simulink model "Caldeira_Controle"  (R2024a)
settings: Solver=ode45  StartTime=0.0  StopTime=260  MaxStep=0.02  RelTol=1e-5
PreLoadFcn:
  | if ~exist('cfg_vap','var') || ~exist('cfg_niv','var'), config_caldeira; end
InitFcn:
  | if ~exist('cfg_vap','var') || ~exist('cfg_niv','var'), config_caldeira; end
settings Model: Creator=Vinicius  LastModifiedBy=Vinicius

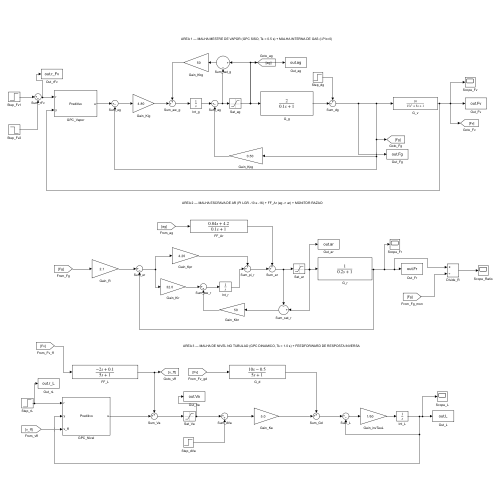
[thumbnail: Simulink's stored preview of the top-level diagram]
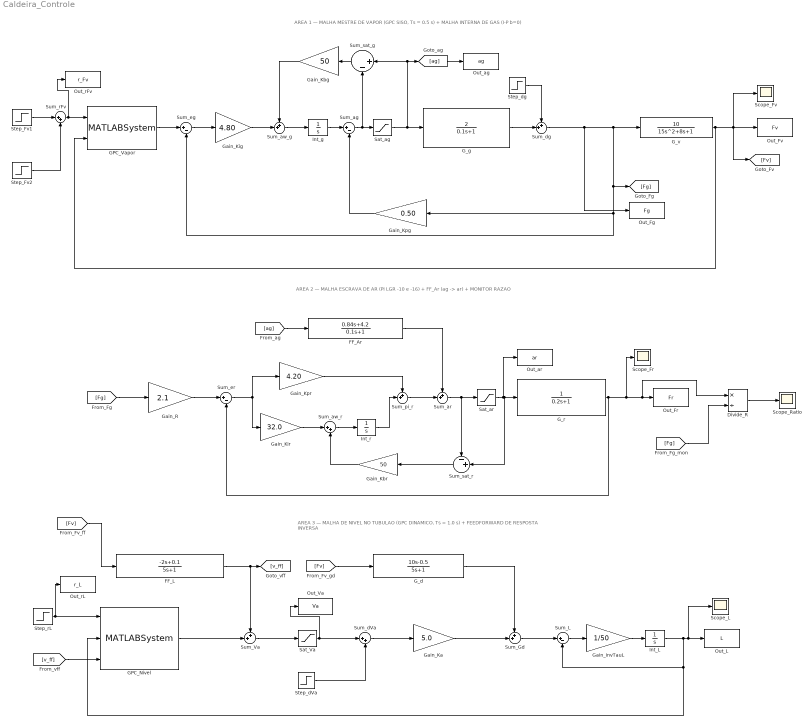
== system Caldeira_Controle ==
  note: AREA 1 — MALHA MESTRE DE VAPOR (GPC SISO, Ts = 0.5 s) + MALHA INTERNA DE GAS (I-P b=0)
  note: AREA 2 — MALHA ESCRAVA DE AR (PI LGR -10 e -16) + FF_Ar (ag -> ar) + MONITOR RAZAO
  note: AREA 3 — MALHA DE NIVEL NO TUBULAO (GPC DINAMICO, Ts = 1.0 s) + FEEDFORWARD DE RESPOSTA INVERSA
  Divide_R : Product  Inputs=*/
  FF_Ar : TransferFcn  Numerator=[0.84 4.2]  Denominator=[0.1 1]
  FF_L : TransferFcn  Numerator=[-2 0.1]  Denominator=[5 1]
  GPC_Nivel : MATLABSystem  System=ControladorPreditivoDin  cfg=cfg_niv
      mask Type: ControladorPreditivoDin
      mask Display:
      | disp('Preditivo');
      | port_label('input',1,'r');
      | port_label('input',2,'y');
      | port_label('input',3,'v_ff');
      | port_label('output',1,'u');
  GPC_Vapor : MATLABSystem  System=ControladorPreditivo  cfg=cfg_vap
      mask Type: ControladorPreditivo
      mask Display:
      | disp('Preditivo');
      | port_label('input',1,'r');
      | port_label('input',2,'y');
      | port_label('output',1,'u');
  G_d : TransferFcn  Numerator=[10 -0.5]  Denominator=[5 1]
  G_g : TransferFcn  Numerator=[2]  Denominator=[0.1 1]
  G_r : TransferFcn  Denominator=[0.2 1]
  G_v : TransferFcn  Numerator=[10]  Denominator=[15 8 1]
  Gain_Ka : Gain  Gain=5.0
  Gain_Kbg : Gain  Gain=50
  Gain_Kbr : Gain  Gain=50
  Gain_Kig : Gain  Gain=4.80
  Gain_Kir : Gain  Gain=32.0
  Gain_Kpg : Gain  Gain=0.50
  Gain_Kpr : Gain  Gain=4.20
  Gain_R : Gain  Gain=2.1
  Gain_invTauL : Gain  Gain=1/50
  Int_L : Integrator  InitialCondition=2.0
  Int_g : Integrator
  Int_r : Integrator
  Out_Fg : ToWorkspace  VariableName=Fg  SampleTime=-1
  Out_Fr : ToWorkspace  VariableName=Fr  SampleTime=-1
  Out_Fv : ToWorkspace  VariableName=Fv  SampleTime=-1
  Out_L : ToWorkspace  VariableName=L  SampleTime=-1
  Out_Va : ToWorkspace  VariableName=Va  SampleTime=-1
  Out_ag : ToWorkspace  VariableName=ag  SampleTime=-1
  Out_ar : ToWorkspace  VariableName=ar  SampleTime=-1
  Out_rFv : ToWorkspace  VariableName=r_Fv  SampleTime=-1
  Out_rL : ToWorkspace  VariableName=r_L  SampleTime=-1
  Sat_Va : Saturate  UpperLimit=1  LowerLimit=0
  Sat_ag : Saturate  UpperLimit=1  LowerLimit=0
  Sat_ar : Saturate  UpperLimit=1  LowerLimit=0
  Scope_Fr : Scope
  Scope_Fv : Scope
  Scope_L : Scope
  Scope_Ratio : Scope
  Step_Fv1 : Step  Time=70  After=2.0  SampleTime=0
  Step_Fv2 : Step  Time=180  After=-0.5  SampleTime=0
  Step_dVa : Step  Time=215  After=0  SampleTime=0
  Step_dg : Step  Time=130  After=0.05  SampleTime=0
  Step_rL : Step  Time=10  Before=2.0  After=2.5  SampleTime=0
  Sum_Gd : Sum  Inputs=++|
  Sum_L : Sum  Inputs=|+-
  Sum_Va : Sum  Inputs=++|
  Sum_ag : Sum  Inputs=|+-
  Sum_ar : Sum  Inputs=++|
  Sum_aw_g : Sum  Inputs=++|
  Sum_aw_r : Sum  Inputs=|++
  Sum_dVa : Sum  Inputs=|++
  Sum_dg : Sum  Inputs=++|
  Sum_eg : Sum  Inputs=|+-
  Sum_er : Sum  Inputs=|+-
  Sum_pi_r : Sum  Inputs=++|
  Sum_rFv : Sum  Inputs=|++
  Sum_sat_g : Sum  Inputs=|+-
  Sum_sat_r : Sum  Inputs=-+|
  wires:
  Step_Fv1/1 -> Sum_rFv/1
  Step_Fv2/1 -> Sum_rFv/2
  Sum_rFv/1 -> GPC_Vapor/1, Out_rFv/1
  GPC_Vapor/1 -> Sum_eg/1
  Sum_eg/1 -> Gain_Kig/1
  Sum_aw_g/1 -> Int_g/1
  Int_g/1 -> Sum_ag/1
  Sum_ag/1 -> Sum_sat_g/2, Sat_ag/1
  G_g/1 -> Sum_dg/2
  Sum_dg/1 -> [Fg], Sum_eg/2, Gain_Kpg/1, G_v/1, Out_Fg/1
  Gain_Kpg/1 -> Sum_ag/2
  G_v/1 -> Scope_Fv/1, Out_Fv/1, [Fv], GPC_Vapor/2
  Sat_ag/1 -> Out_ag/1, G_g/1, [ag], Sum_sat_g/1
  Step_dg/1 -> Sum_dg/1
  Sum_sat_g/1 -> Gain_Kbg/1
  Gain_Kig/1 -> Sum_aw_g/2
  Gain_Kbg/1 -> Sum_aw_g/1
  [Fg] -> Gain_R/1
  Gain_R/1 -> Sum_er/1
  Sum_er/1 -> Gain_Kpr/1, Gain_Kir/1
  Sum_aw_r/1 -> Int_r/1
  Gain_Kpr/1 -> Sum_pi_r/1
  Int_r/1 -> Sum_pi_r/2
  [ag] -> FF_Ar/1
  FF_Ar/1 -> Sum_ar/1
  Sum_pi_r/1 -> Sum_ar/2
  Sum_ar/1 -> Sum_sat_r/1, Sat_ar/1
  Sat_ar/1 -> Sum_sat_r/2, G_r/1, Out_ar/1
  G_r/1 -> Out_Fr/1, Divide_R/1, Scope_Fr/1, Sum_er/2
  [Fg] -> Divide_R/2
  Divide_R/1 -> Scope_Ratio/1
  Sum_sat_r/1 -> Gain_Kbr/1
  Gain_Kir/1 -> Sum_aw_r/1
  Gain_Kbr/1 -> Sum_aw_r/2
  [Fv] -> FF_L/1
  FF_L/1 -> Sum_Va/1, [v_ff]
  Step_rL/1 -> GPC_Nivel/1, Out_rL/1
  [v_ff] -> GPC_Nivel/3
  Sum_Va/1 -> Sat_Va/1
  Step_dVa/1 -> Sum_dVa/2
  Sum_dVa/1 -> Gain_Ka/1
  [Fv] -> G_d/1
  G_d/1 -> Sum_Gd/1
  Sum_Gd/1 -> Sum_L/1
  Sum_L/1 -> Gain_invTauL/1
  Gain_invTauL/1 -> Int_L/1
  Int_L/1 -> Out_L/1, Scope_L/1, Sum_L/2, GPC_Nivel/2
  GPC_Nivel/1 -> Sum_Va/2
  Sat_Va/1 -> Sum_dVa/1, Out_Va/1
  Gain_Ka/1 -> Sum_Gd/2
